simulink model "UAM_Hexa_PD_Obs_SinSimscape_triste"  (R2026a)
settings: Solver=ode4  StopTime=tf  FixedStep=0.01
values from neighbouring files (symbols this model uses):
  ArmConstants = struct('l1_dim', l1_dim,                        'l2_dim', l2_dim,                        'Hexa_to_joint_L', L,                        'Mass1', ml1,                        'Mass2', ml2,                        'Inertia1', Hl1,                        'Inertia2', Hl2,                        'MC1', c1,                        'MC2', c2,                        'Servos', Servos)    [init_model.m]    (also in init_var.m)
  HexaConstants = struct('Mass', mb,                         'Inertia', J ,                         'allo', allo,                          'invallo', invallo,                         'kT', kT)    [init_model.m]    (also in init_var.m)
  Observer = struct('E1', E1 ,     'E2', E2 ,     'E3', E3 ,     'E4', E4 ,     'MU1', MU1 ,     'MU2', MU2 ,     'MU3', MU3 ,     'alpha', alpha ,     'beta', beta)    [init_model.m]    (also in init_var.m)
  PID = InitController()    [init_model.m]    (also in init_var.m)
settings Model: Creator=Carlos Fabian  LastModifiedBy=Carlos Fabian
settings ExplorerConfigSet: InternalSimMechanicsExplorerSettings=|
  | <ExplorerConfiguration>
  | 
  |   <canonicalview>default</canonicalview>
  | 
  |   <TilePanel>
  |     <TileInfo>
  |       <Tiles Columns="1" Count="1" Height="513" Rows="1" Width="774">
  |         <Row Weight="1"/>
  |         <Column Weight="1"/>
  |         <Tile Height="1" Width="1" X="0" Y="0"/>
  |       </Tiles>
  |     </TileInfo>
  |     <SceneInfo>
  |       <SceneViewer>
  |         <IsThisViewStd>
  |           <IsStandardView>off</IsStandardView>
  |           <StandardViewName>Front</StandardViewName>
  |         </IsThisViewStd>
  |         <BGColor>
  |           <R>1</R>
  |           <G>1</G>
  |           <B>1</B>
  |           <A>1</A>
  |         </BGColor>
  |         <Camera>
  |           <DoPerspective>off</DoPerspective>
  |           <Position>
  |             <X>16.201091586104312</X>
  |             <Y>-16.65504514146788</Y>
  |             <Z>17.087073385082522</Z>
  |           </Position>
  |           <Center>
  |             <X>-0.25720946651222221</X>
  |             <Y>-0.19674408885134653</Y>
  |             <Z>0.62877233246599318</Z>
  |           </Center>
  |           <Up>
  |             <X>-0.40824829046386302</X>
  |             <Y>0.40824829046386302</Y>
  |             <Z>0.81649658092772615</Z>
  |           </Up>
  |           <XLim>2.5491252053936631</XLim>
  |           <YLim>2.5491252053936631</YLim>
  |           <ViewLimDist>0.01</ViewLimDist>
  |         </Camera>
  |       </SceneViewer>
  |     </SceneInfo>
  |   </TilePanel>
  | 
  |   <MechEditorPanel>
  |     <GfxPanelCameraMap/>
  |     <Cameras/>
  |     <VideoCreator>
  |       <IncludeTiles>All</IncludeTiles>
  |       <IncludeTime>on</IncludeTime>
  |       <IncludeWorldFrame>off</IncludeWorldFrame>
  |       <PlaybackSpeedRatio>8</PlaybackSpeedRatio>
  |       <FrameRate>24</FrameRate>
  |       <FrameSize>auto</FrameSize>
  |       <VideoFormat>MotionJPEGAVI</VideoFormat>
  |     </VideoCreator>
  |   </MechEditorPanel>
  | 
  |   <PlaybackSettings>
  |     <PlaybackSpeedFactor>16</PlaybackSpeedFactor>
  |   </PlaybackSettings>
  | 
  | </ExplorerConfiguration>

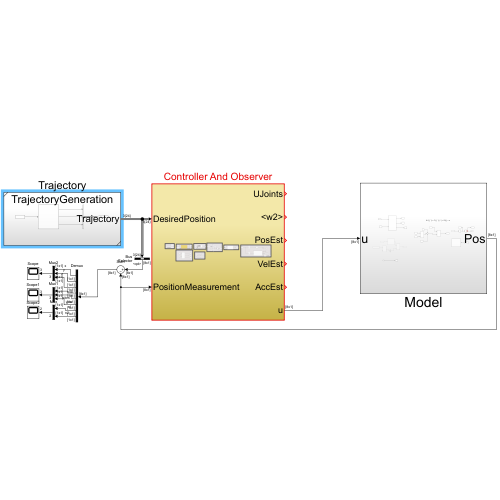
[thumbnail: Simulink's stored preview of the top-level diagram]
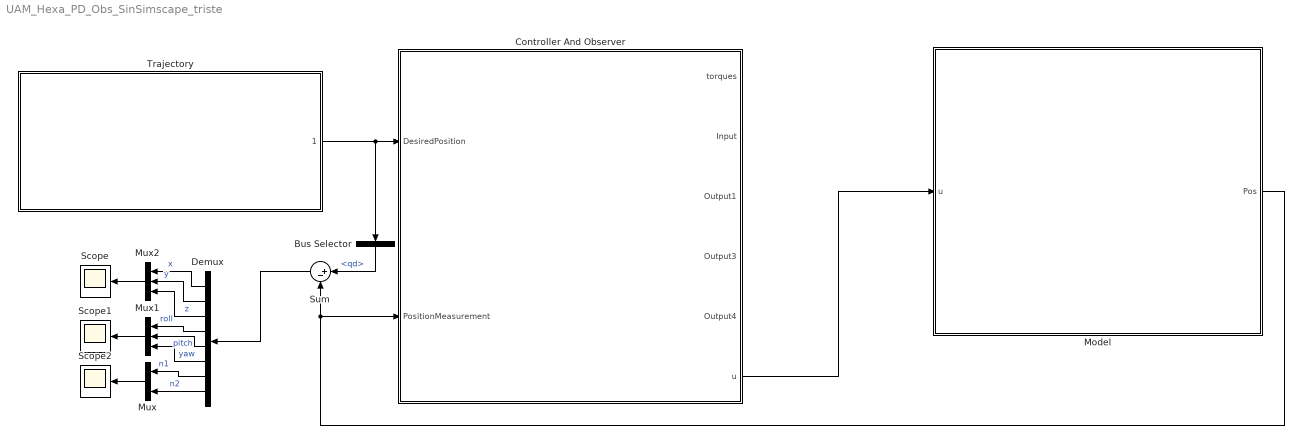
== system UAM_Hexa_PD_Obs_SinSimscape_triste ==
  Bus Selector : BusSelector  OutputSignals=qd
  Controller And Observer : Subsystem  TreatAsAtomicUnit=on
  Demux : Demux  Outputs=8
  Model : Subsystem
  Mux : Mux  Inputs=2
  Mux1 : Mux  Inputs=3
  Mux2 : Mux  Inputs=3
  Scope : Scope
      settings: ActiveDisplayYMinimum=-0.10157502958143397  ActiveDisplayYMaximum=0.28934279536970853
  Scope1 : Scope
      settings: ActiveDisplayYMinimum=-0.00621682249259307  ActiveDisplayYMaximum=0.012057716917689382
  Scope2 : Scope
      settings: ActiveDisplayYMinimum=-0.033824684374711443  ActiveDisplayYMaximum=0.027672278232653655  DataLoggingVariableName=ScopeData2
  Sum : Sum  Inputs=|+-
  Trajectory : Subsystem  ReferencedSubsystem=TrajectoryGeneration
  wires:
  Trajectory/1 -> Bus Selector/1, Controller And Observer/1(DesiredPosition)
  Model/1(Pos) -> Controller And Observer/2(PositionMeasurement), Sum/2
  Bus Selector/1 -> Sum/1  "<qd>"
  Sum/1 -> Demux/1
  Mux2/1 -> Scope/1
  Mux1/1 -> Scope1/1
  Mux/1 -> Scope2/1
  Demux/1 -> Mux2/1  "x"
  Demux/2 -> Mux2/2  "y"
  Demux/3 -> Mux2/3  "z"
  Demux/4 -> Mux1/1  "roll"
  Demux/5 -> Mux1/2  "pitch"
  Demux/6 -> Mux1/3  "yaw"
  Demux/7 -> Mux/1  "n1"
  Demux/8 -> Mux/2  "n2"
  Controller And Observer/6(u) -> Model/1(u)

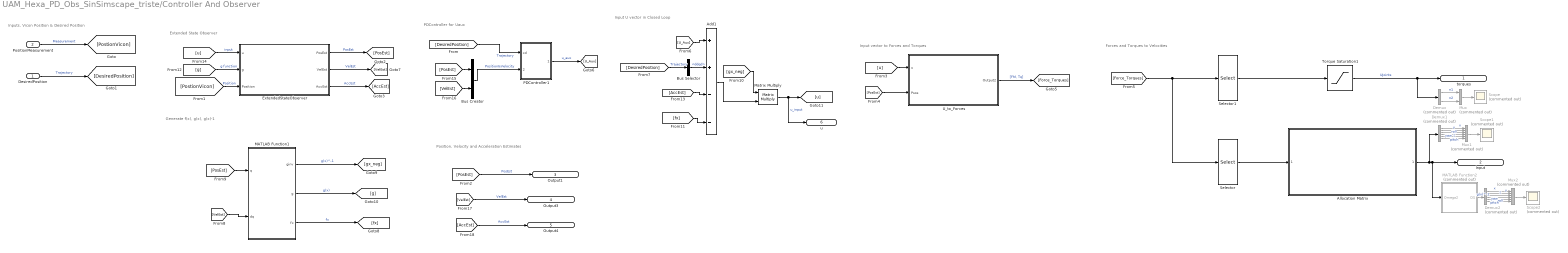
== system UAM_Hexa_PD_Obs_SinSimscape_triste/Controller And Observer ==
  note: Position, Velocity and Acceleration Estimates
  note: Input vector to Forces and Torques
  note: Forces and Torques to Velocities
  note: Extended State Observer
  note: Input U vector in Closed Loop
  note: Generate f(x), g(x), g(x)-1
  note: PDController for Uaux
  note: Inputs, Vicon Position & Desired Position
  DesiredPosition : Inport  SampleTime=0.01
  PositionMeasurement : Inport  Port=2  SampleTime=0.01
  Add1 : Sum  Inputs=++--
  Allocation Matrix : Subsystem  ReferencedSubsystem=FromFMtoOmega2
  Bus Creator : BusCreator  Inputs=2
  Bus Selector : BusSelector  OutputSignals=ddqd
  Demux : Demux  Commented=on  Outputs=2
  Demux1 : Demux  Commented=on  Outputs=6
  Demux2 : Demux  Commented=on  Outputs=6
  ExtendedStateObserver : Subsystem
  MATLAB Function1 : MATLAB Function  TreatAsAtomicUnit=on
  MATLAB Function2 : MATLAB Function  Commented=on  TreatAsAtomicUnit=on
  Matrix Multiply : Product  Multiplication=Matrix(*)
  Mux : Mux  Commented=on  Inputs=2
  Mux1 : Mux  Commented=on  Inputs=6
  Mux2 : Mux  Commented=on  Inputs=6
  PDController1 : Subsystem
  Scope : Scope  Commented=on
      settings: ActiveDisplayYMinimum=-0.14254925702084698  ActiveDisplayYMaximum=0.588439761419796  DataLoggingVariableName=ScopeData3
  Scope1 : Scope  Commented=on
      settings: ActiveDisplayYMinimum=281288.18904371274  ActiveDisplayYMaximum=661748.11016186653  DataLoggingVariableName=ScopeData4
  Scope2 : Scope  Commented=on
      settings: ActiveDisplayYMinimum=0.68328386023492  ActiveDisplayYMaximum=1.0389756799900849  DataLoggingVariableName=ScopeData5
  Selector : Selector  InputPortWidth=8  IndexOptions=Index vector (dialog)  Indices=1:6  OutputSizes=1
  Selector1 : Selector  InputPortWidth=8  IndexOptions=Index vector (dialog)  Indices=7:8  OutputSizes=1
  Torque Saturation1 : Saturate  UpperLimit=ArmConstants.Servos.T1max  LowerLimit=-ArmConstants.Servos.T1max
  U_to_Forces : Subsystem
  torques : Outport  SampleTime=0.01
  Input : Outport  Port=2  SampleTime=0.01
  Output1 : Outport  Port=3
  Output3 : Outport  Port=4
  Output4 : Outport  Port=5
  u : Outport  Port=6  SampleTime=0.01
  wires:
  [PostionVicon] -> ExtendedStateObserver/3(Position)  "Position"
  [DesiredPosition] -> PDController1/1(xd)  "Trajectory"
  U_to_Forces/1(Output2) -> [Force_Torques]  "[FM, Tq]"
  ExtendedStateObserver/1(PosEst) -> [PosEst]  "PosEst"
  PositionMeasurement/1 -> [PostionVicon]  "Measurement"
  DesiredPosition/1 -> [DesiredPosition]  "Trajectory"
  Bus Creator/1 -> PDController1/2(q_hat1)  "Position&Velocity"
  ExtendedStateObserver/3(AccEst) -> [AccEst]  "AccEst"
  ExtendedStateObserver/2(VelEst) -> [VelEst]  "VelEst"
  [PosEst] -> U_to_Forces/2(Psos)
  Selector1/1 -> Torque Saturation1/1
  [Force_Torques] -> Selector/1, Selector1/1
  Selector/1 -> Allocation Matrix/1
  Torque Saturation1/1 -> Demux/1, torques/1  "UJoints"
  Allocation Matrix/1 -> Demux1/1, Input/1, MATLAB Function2/1(Omega2)
  PDController1/1(Output) -> [U_Aux]  "u_aux"
  MATLAB Function1/1(ginv) -> [gx_neg]  "g(x)^-1"
  MATLAB Function1/3(fx) -> [fx]  "fx"
  [VelEst] -> MATLAB Function1/2(dq)
  [PosEst] -> MATLAB Function1/1(q)
  [fx] -> Add1/4
  Add1/1 -> Matrix Multiply/2
  [gx_neg] -> Matrix Multiply/1
  [U_Aux] -> Add1/1
  [DesiredPosition] -> Bus Selector/1  "Trajectory"
  Bus Selector/1 -> Add1/2  "<ddqd>"
  [AccEst] -> Add1/3
  MATLAB Function1/2(g) -> [g]  "g(x)"
  [g] -> ExtendedStateObserver/2(g)  "g function"
  [u] -> ExtendedStateObserver/1(u)  "input"
  [PosEst] -> Bus Creator/1
  [VelEst] -> Bus Creator/2
  [u] -> U_to_Forces/1(u)
  [PosEst] -> Output1/1  "PosEst"
  [VelEst] -> Output3/1  "VelEst"
  [AccEst] -> Output4/1  "AccEst"
  Matrix Multiply/1 -> u/1, [u]  "u_input"
  Demux/1 -> Mux/1  "n1"
  Demux/2 -> Mux/2  "n2"
  Mux/1 -> Scope/1
  Mux1/1 -> Scope1/1
  Demux1/1 -> Mux1/1  "x"
  Demux1/2 -> Mux1/2  "y"
  Demux1/3 -> Mux1/3  "z"
  Demux1/4 -> Mux1/4  "roll"
  Demux1/5 -> Mux1/5  "pitch"
  Demux1/6 -> Mux1/6  "yaw"
  Demux2/1 -> Mux2/1  "x"
  Demux2/3 -> Mux2/3  "z"
  Demux2/4 -> Mux2/4  "roll"
  Demux2/6 -> Mux2/6  "yaw"
  Demux2/5 -> Mux2/5  "pitch"
  Mux2/1 -> Scope2/1
  Demux2/2 -> Mux2/2  "y"
  MATLAB Function2/1(DS) -> Demux2/1  "g(x)^-1"

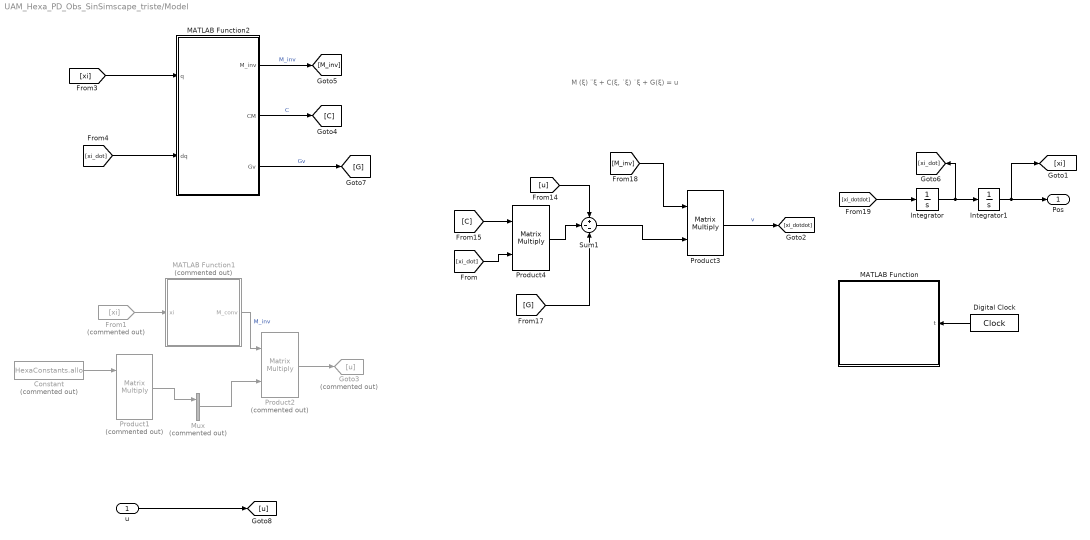
== system UAM_Hexa_PD_Obs_SinSimscape_triste/Model ==
  note: M (ξ) ¨ξ + C(ξ, ˙ξ) ˙ξ + G(ξ) = u
  u : Inport
  Constant : Constant  Commented=on  Value=HexaConstants.allo
  Digital Clock : DigitalClock  SampleTime=0.01
  From1 : From  Commented=on  GotoTag=xi
  Goto3 : Goto  Commented=on  GotoTag=u
  Integrator : Integrator  InitialCondition=zeros(8,1)
  Integrator1 : Integrator  InitialCondition=zeros(8,1)
  MATLAB Function : MATLAB Function  TreatAsAtomicUnit=on
  MATLAB Function1 : MATLAB Function  Commented=on  TreatAsAtomicUnit=on
  MATLAB Function2 : MATLAB Function  TreatAsAtomicUnit=on
  Mux : Mux  Commented=on  Inputs=2
  Product1 : Product  Commented=on  Multiplication=Matrix(*)
  Product2 : Product  Commented=on  Multiplication=Matrix(*)
  Product3 : Product  Multiplication=Matrix(*)
  Product4 : Product  Multiplication=Matrix(*)
  Sum1 : Sum  Inputs=+--
  Pos : Outport  SampleTime=0.01
  wires:
  Integrator1/1 -> [xi], Pos/1
  [u] -> Sum1/1
  [C] -> Product4/1
  [G] -> Sum1/3
  Sum1/1 -> Product3/2
  [M_inv] -> Product3/1
  Product4/1 -> Sum1/2
  Product3/1 -> [xi_dotdot]  "v"
  [xi_dotdot] -> Integrator/1
  Integrator/1 -> [xi_dot], Integrator1/1
  Digital Clock/1 -> MATLAB Function/1(t)
  MATLAB Function2/3(Gv) -> [G]  "Gv"
  MATLAB Function2/2(CM) -> [C]  "C"
  MATLAB Function2/1(M_inv) -> [M_inv]  "M_inv"
  [xi] -> MATLAB Function2/1(q)
  [xi_dot] -> MATLAB Function2/2(dq)
  [xi_dot] -> Product4/2
  u/1 -> [u]
  Constant/1 -> Product1/1
  Product1/1 -> Mux/1
  Mux/1 -> Product2/2
  Product2/1 -> Goto3/1
  MATLAB Function1/1(M_conv) -> Product2/1  "M_inv"
  From1/1 -> MATLAB Function1/1(xi)

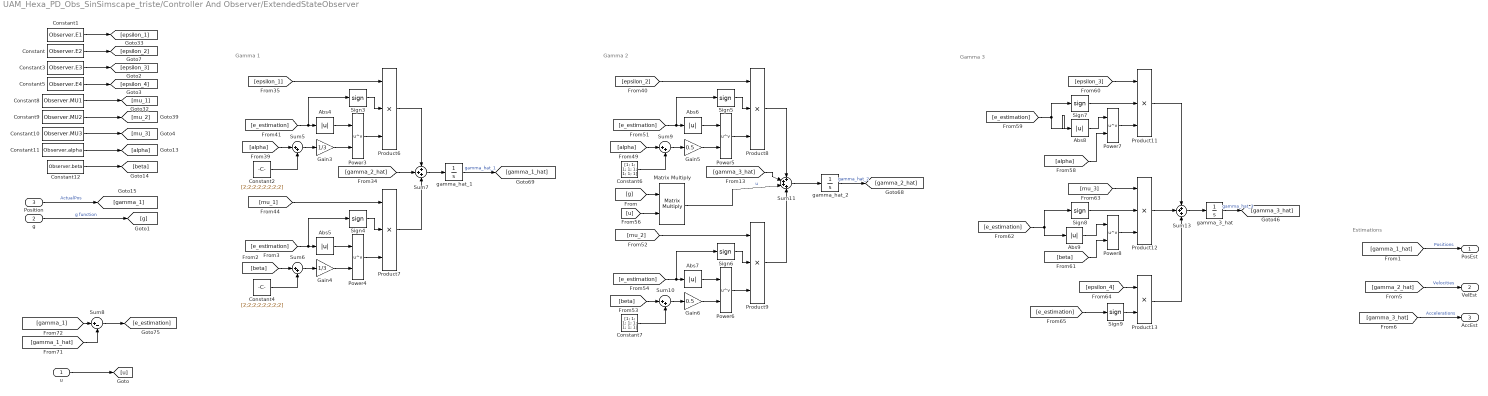
== system UAM_Hexa_PD_Obs_SinSimscape_triste/Controller And Observer/ExtendedStateObserver ==
  note: Estimations
  note: Gamma 3
  note: Gamma 2
  note: Gamma 1
  u : Inport  SampleTime=0.01
  g : Inport  Port=2  SampleTime=0.01
  Position : Inport  Port=3  SampleTime=0.01
  Abs{4..9} (6 alike) : Abs  SaturateOnIntegerOverflow=off
  Constant : Constant  Value=Observer.E2
  Constant1 : Constant  Value=Observer.E1
  Constant10 : Constant  Value=Observer.MU3
  Constant11 : Constant  Value=Observer.alpha
  Constant12 : Constant  Value=Observer.beta
  Constant2 : Constant  Value=[2;2;2;2;2;2;2;2]
  Constant3 : Constant  Value=Observer.E3
  Constant4 : Constant  Value=[2;2;2;2;2;2;2;2]
  Constant5 : Constant  Value=Observer.E4
  Constant6 : Constant  Value=[1; 1; 1; 1; 1; 1; 1; 1]
  Constant7 : Constant  Value=[1; 1; 1; 1; 1; 1; 1; 1]
  Constant8 : Constant  Value=Observer.MU1
  Constant9 : Constant  Value=Observer.MU2
  Gain3 : Gain  Gain=1/3
  Gain4 : Gain  Gain=1/3
  Gain5 : Gain  Gain=0.5
  Gain6 : Gain  Gain=0.5
  Matrix Multiply : Product  Multiplication=Matrix(*)
  Power{3..8} (6 alike) : Math  Operator=pow
  Product{6..9,11..12} (6 alike) : Product  Inputs=3
  Product13 : Product
  Sign{3..9} (7 alike) : Signum
  Sum{5..6,9..10} (4 alike) : Sum  Inputs=|++
  Sum11 : Sum  Inputs=++++
  Sum13 : Sum  Inputs=+++
  Sum7 : Sum  Inputs=+++
  Sum8 : Sum  Inputs=|+-
  gamma_3_hat : Integrator  InitialCondition=[0; 0; -9.81; 0; 0; 0; 0; 0]
  gamma_hat_1 : Integrator  InitialCondition=[0; 0; 0.24; 0; 0; 0; 0; 0]
  gamma_hat_2 : Integrator  InitialCondition=zeros(8,1)
  PosEst : Outport  SampleTime=0.01
  VelEst : Outport  Port=2  SampleTime=0.01
  AccEst : Outport  Port=3  SampleTime=0.01
  wires:
  Constant11/1 -> [alpha]
  [beta] -> Sum10/1
  [e_estimation] -> Sign8/1, Abs9/1
  Power7/1 -> Product11/3
  Matrix Multiply/1 -> Sum11/3  "u"
  Constant12/1 -> [beta]
  [e_estimation] -> Abs8/1, Sign7/1
  [gamma_1_hat] -> PosEst/1  "Positions"
  Power8/1 -> Product12/3
  Constant4/1 -> Sum6/2
  [alpha] -> Sum5/1
  Product6/1 -> Sum7/1
  Abs8/1 -> Power7/1
  Power5/1 -> Product8/3
  [gamma_1] -> Sum8/1
  [e_estimation] -> Sign6/1, Abs7/1
  [epsilon_2] -> Product8/1
  Sum11/1 -> gamma_hat_2/1
  Constant10/1 -> [mu_3]
  Gain5/1 -> Power5/2
  [e_estimation] -> Sign3/1, Abs4/1
  Abs5/1 -> Power4/1
  Sum13/1 -> gamma_3_hat/1
  Abs7/1 -> Power6/1
  Product9/1 -> Sum11/4
  [epsilon_1] -> Product6/1
  Constant7/1 -> Sum10/2
  [epsilon_3] -> Product11/1
  Sum9/1 -> Gain5/1
  Sum6/1 -> Gain4/1
  [e_estimation] -> Sign5/1, Abs6/1
  u/1 -> [u]
  [mu_3] -> Product12/1
  Sign6/1 -> Product9/2
  Sum7/1 -> gamma_hat_1/1
  Sign8/1 -> Product12/2
  [alpha] -> Power7/2
  [epsilon_4] -> Product13/1
  [gamma_3_hat] -> Sum11/2
  [mu_1] -> Product7/1
  Sign3/1 -> Product6/2
  gamma_hat_2/1 -> [gamma_2_hat]  "gamma_hat_2"
  Constant/1 -> [epsilon_2]
  [mu_2] -> Product9/1
  Product11/1 -> Sum13/1
  [gamma_1_hat] -> Sum8/2
  Sign4/1 -> Product7/2
  Product7/1 -> Sum7/3
  Constant9/1 -> [mu_2]
  Constant1/1 -> [epsilon_1]
  Constant6/1 -> Sum9/2
  Sign5/1 -> Product8/2
  [beta] -> Power8/2
  Constant2/1 -> Sum5/2
  Gain6/1 -> Power6/2
  Gain3/1 -> Power3/2
  Power6/1 -> Product9/3
  Position/1 -> [gamma_1]  "ActualPos"
  Constant5/1 -> [epsilon_4]
  Constant3/1 -> [epsilon_3]
  Product13/1 -> Sum13/3
  gamma_hat_1/1 -> [gamma_1_hat]  "gamma_hat_1"
  Sum5/1 -> Gain3/1
  Power3/1 -> Product6/3
  Power4/1 -> Product7/3
  Sum10/1 -> Gain6/1
  [gamma_2_hat] -> Sum7/2
  Sign7/1 -> Product11/2
  [beta] -> Sum6/1
  [e_estimation] -> Sign4/1, Abs5/1
  [e_estimation] -> Sign9/1
  Product8/1 -> Sum11/1
  Sign9/1 -> Product13/2
  Abs9/1 -> Power8/1
  [alpha] -> Sum9/1
  gamma_3_hat/1 -> [gamma_3_hat]  "gamma_hat_3"
  Sum8/1 -> [e_estimation]
  Gain4/1 -> Power4/2
  Constant8/1 -> [mu_1]
  Product12/1 -> Sum13/2
  g/1 -> [g]  "g function"
  Abs6/1 -> Power5/1
  Abs4/1 -> Power3/1
  [gamma_3_hat] -> AccEst/1  "Accelerations"
  [gamma_2_hat] -> VelEst/1  "Velocities"
  [g] -> Matrix Multiply/1
  [u] -> Matrix Multiply/2

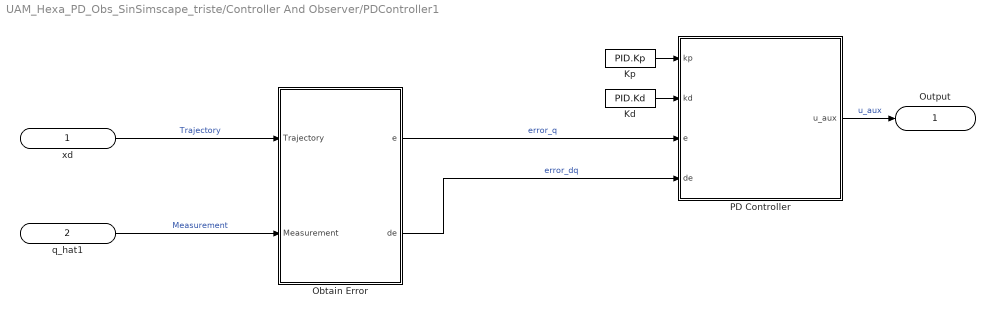
== system UAM_Hexa_PD_Obs_SinSimscape_triste/Controller And Observer/PDController1 ==
  xd : Inport
  q_hat1 : Inport  Port=2
  Kd : Constant  Value=PID.Kd
  Kp : Constant  Value=PID.Kp
  Obtain Error : Subsystem
  PD Controller : MATLAB Function  TreatAsAtomicUnit=on
  Output : Outport
  wires:
  xd/1 -> Obtain Error/1(Trajectory)  "Trajectory"
  q_hat1/1 -> Obtain Error/2(Measurement)  "Measurement"
  Obtain Error/1(e) -> PD Controller/3(e)  "error_q"
  Obtain Error/2(de) -> PD Controller/4(de)  "error_dq"
  Kp/1 -> PD Controller/1(kp)
  Kd/1 -> PD Controller/2(kd)
  PD Controller/1(u_aux) -> Output/1  "u_aux"

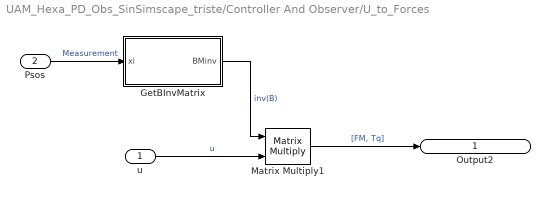
== system UAM_Hexa_PD_Obs_SinSimscape_triste/Controller And Observer/U_to_Forces ==
  u : Inport
  Psos : Inport  Port=2
  GetBInvMatrix : MATLAB Function  TreatAsAtomicUnit=on
  Matrix Multiply1 : Product  Multiplication=Matrix(*)
  Output2 : Outport
  wires:
  Psos/1 -> GetBInvMatrix/1(xi)  "Measurement"
  u/1 -> Matrix Multiply1/2  "u"
  Matrix Multiply1/1 -> Output2/1  "[FM, Tq]"
  GetBInvMatrix/1(BMinv) -> Matrix Multiply1/1  "inv(B)"

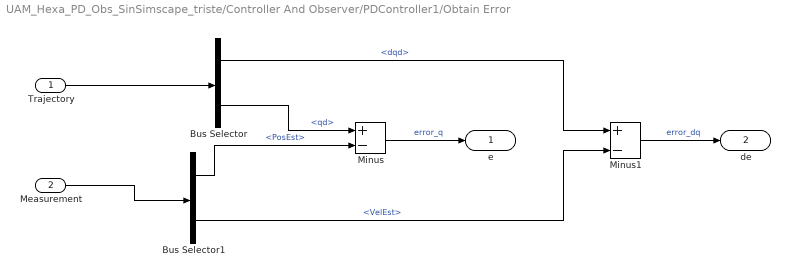
== system UAM_Hexa_PD_Obs_SinSimscape_triste/Controller And Observer/PDController1/Obtain Error ==
  Trajectory : Inport
  Measurement : Inport  Port=2
  Bus Selector : BusSelector  OutputSignals=dqd,qd
  Bus Selector1 : BusSelector  OutputSignals=PosEst,VelEst
  Minus : Sum  Inputs=+-
  Minus1 : Sum  Inputs=+-
  e : Outport
  de : Outport  Port=2
  wires:
  Bus Selector1/1 -> Minus/2  "<PosEst>"
  Bus Selector1/2 -> Minus1/2  "<VelEst>"
  Measurement/1 -> Bus Selector1/1
  Trajectory/1 -> Bus Selector/1
  Bus Selector/1 -> Minus1/1  "<dqd>"
  Bus Selector/2 -> Minus/1  "<qd>"
  Minus/1 -> e/1  "error_q"
  Minus1/1 -> de/1  "error_dq"

== matlab function UAM_Hexa_PD_Obs_SinSimscape_triste/Model/MATLAB Function2 ==
  data: q input; dq input; HexaConstants parameter; M_inv output; CM output; Gv output; ArmConstants parameter
function [M_inv, CM, Gv] = Get_DCG_Hexa(q, dq, HexaConstants, ArmConstants)

DM = DMatrix(q, HexaConstants, ArmConstants);
CM = CMatrix(q, dq, HexaConstants, ArmConstants);
Gv = GVector(q, HexaConstants, ArmConstants);

M_inv = inv(DM);

end

== matlab function UAM_Hexa_PD_Obs_SinSimscape_triste/Controller And Observer/PDController1/PD Controller ==
  data: kp input; kd input; u_aux output; e input; de input
function u_aux = pd_cont(kp, kd, e, de)


kp_m = [kp(1) 0       0     0     0       0     0     0;
        0     kp(2)   0     0     0       0     0     0;
        0     0       kp(3) 0     0       0     0     0;
        0     0       0     kp(4) 0       0     0     0;
        0     0       0     0     kp(5)   0     0     0;
        0     0       0     0     0       kp(6) 0     0;
        0     0       0     0     0       0     kp(7) 0;
        0     0       0     0     0       0     0     kp(8)];

kd_m = [kd(1) 0       0     0     0       0     0     0;
        0     kd(2)   0     0     0       0     0     0;
        0     0       kd(3) 0     0       0     0     0;
        0     0       0     kd(4) 0       0     0     0;
        0     0       0     0     kd(5)   0     0     0;
        0     0       0     0     0       kd(6) 0     0;
        0     0       0     0     0       0     kd(7) 0;
        0     0       0     0     0       0     0     kd(8)];


%v = ddP + kp_m * e + kd_m * de;
u_aux = kp_m * e + kd_m * de;
%v = ddP;

end

== matlab function UAM_Hexa_PD_Obs_SinSimscape_triste/Model/MATLAB Function1 ==
  data: xi input; M_conv output
function M_conv  = Get_DCG_Hexa(xi)

phi = xi(4);
theta = xi(5);
psi = xi(6);

C_phi = cos(phi);
S_phi = sin(phi);
    
C_theta = cos(theta);
S_theta = sin(theta);
    
C_psi = cos(psi);
S_psi = sin(psi);

Rb = [
C_psi*C_theta,  C_psi*S_phi*S_theta - C_phi*S_psi,  S_phi*S_psi + C_phi*C_psi*S_theta;
C_theta*S_psi,  C_phi*C_psi + S_psi*S_theta*S_phi, -C_psi*S_phi + S_psi*S_theta*C_phi;
-S_theta,        C_theta*S_phi,                      S_theta*C_phi
];

W = [
1,       0,        -S_theta;
0,   C_phi,  C_theta*S_phi;
0,  -S_phi,  C_theta*C_phi
];

w_inv = inv(W);

M_conv = [Rb, zeros(3,3), zeros(3,2);
    zeros(3,3), w_inv, zeros(3,2);
    zeros(2,3), zeros(2,3), eye(2)];

end

== matlab function UAM_Hexa_PD_Obs_SinSimscape_triste/Model/MATLAB Function ==
  data: t input; PickObj parameter
function GetPickObj(t, PickObj)

Times = PickObj.Time;

if length(Times) == 2
    cond = t <= Times(1) || t >= Times(2);
else
    cond = t <= Times(1);
end

if ~cond
    m = PickObj.Mass;
    r = PickObj.Radius;
    I1 = 2/5*m*r^2;
    I = diag([I1, I1, I1]);
else
    m = 0;
    I = zeros(3, 3);
end

end

== matlab function UAM_Hexa_PD_Obs_SinSimscape_triste/Controller And Observer/MATLAB Function2 ==
  data: Omega2 input; DS output
function DS = calcular_DS(Omega2)
    p2 = 8.8803e-4;
    p1 = 0.1431;
    p0 = 1094;
    % DS = p2 .* Omega2 + p1 .* sqrt(Omega2) + p0;
    DS = (p2 .* Omega2 + p1 .* sqrt(Omega2) + p0)/2000;
end

== matlab function UAM_Hexa_PD_Obs_SinSimscape_triste/Controller And Observer/MATLAB Function1 ==
  data: q input; dq input; HexaConstants parameter; ginv output; g output; fx output; ArmConstants parameter
function [ginv, g, fx] = Get_DCG_Hexa(q, dq, HexaConstants, ArmConstants)

DM = DMatrix(q, HexaConstants, ArmConstants);
CM = CMatrix(q, dq, HexaConstants, ArmConstants);
Gv = GVector(q, HexaConstants, ArmConstants);

g = inv(DM);
ginv = DM;

fx = DM\( -CM*dq - Gv );

end

== matlab function UAM_Hexa_PD_Obs_SinSimscape_triste/Controller And Observer/U_to_Forces/GetBInvMatrix ==
  data: xi input; BMinv output
function BMinv = GetBInvMatrix(xi)

% phi = xi(4);
% th  = xi(5);
% psi = xi(6);
% 
% BM1=[cos(phi)*cos(th),-cos(phi)*sin(psi)+cos(psi)*sin(phi)*sin(th), ...
%     sin(phi)*sin(psi)+cos(phi)*cos(psi)*sin(th),0,0,0;...
%     cos(th)*sin(psi), cos(phi)*cos(psi)+sin(phi)*sin(psi)*sin(th),...
%     -cos(psi)*sin(phi)+cos(phi)*sin(psi)*sin(phi),0,0,0;...
%     -sin(th),cos(th)*sin(psi),cos(phi)*cos(th),0,0,0;...
%     0,0,0,1,sin(phi)*tan(th),cos(phi)*tan(th);...
%     0,0,0,0,cos(phi),-sin(phi);0,0,0,0,sec(th)*sin(phi),cos(phi)*sec(th)];

BM1 = BMatrix(xi);

BM = blkdiag(BM1, eye(2,2));

BMinv = inv(BM);

end
